simulink model "Earthquake_Undamped"  (R2026a)
settings: Solver=VariableStepAuto  StopTime=20

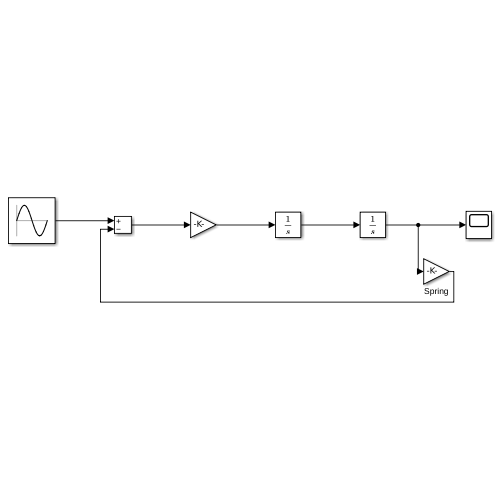
[thumbnail: Simulink's stored preview of the top-level diagram]
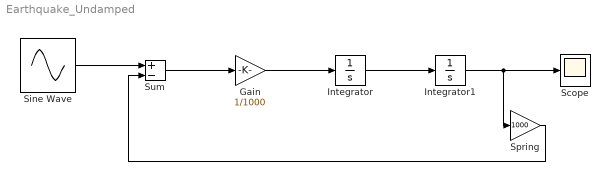
== system Earthquake_Undamped ==
  Gain : Gain  Gain=1/1000
  Integrator : Integrator
  Integrator1 : Integrator
  Scope : Scope
      settings: ActiveDisplayYMinimum=-0.62466762030279943  ActiveDisplayYMaximum=0.62321764758307
  Sine Wave : Sin  Amplitude=1000  Frequency=3  SampleTime=0
  Spring : Gain  Gain=1000
  Sum : Sum  Inputs=+-
  wires:
  Gain/1 -> Integrator/1
  Integrator/1 -> Integrator1/1
  Integrator1/1 -> Spring/1, Scope/1
  Spring/1 -> Sum/2
  Sum/1 -> Gain/1
  Sine Wave/1 -> Sum/1
